simulink model "Regelkreis_T4_restored_from_autosave"  (R2025b)
settings: Solver=ode3  StartTime=0.0  StopTime=3  FixedStep=0.02  RelTol=1e-3
model workspace (MAT data in the model file):
  K_I = 1
  T_1 = [1 1]
settings Model: ExtModeTrigDuration=100  Creator=ofm31594  LastModifiedBy=janis

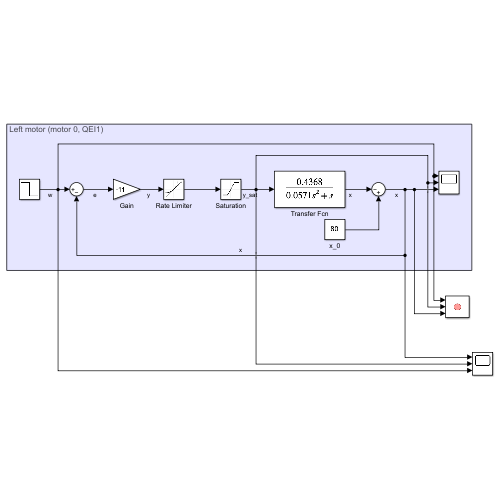
[thumbnail: Simulink's stored preview of the top-level diagram]
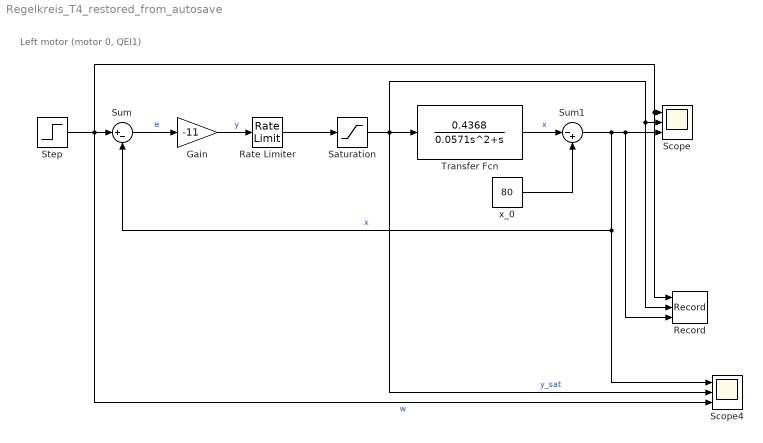
== system Regelkreis_T4_restored_from_autosave ==
  note: Left motor (motor 0, QEI1)
  Gain : Gain  Gain=-11
  Rate Limiter : RateLimiter  RisingSlewLimit=4/0.02  FallingSlewLimit=-20000  SampleTimeMode=inherited
  Record : Record  NumPorts=3.0  FileSettingsInternal="{\"entries\":[{\"content\":{\"excelSettings\":{\"content\":{},\"type\":\"Streamout.ExcelSettings\"},\"parquetSettings\":{\"content\":{},\"type\":\"Streamout.ParquetSettings\"}},\"type\":\"Streamout.FileSettingStorage\",\"uuid\":\"\"}],\"packageUris\":[\"http:\\/\\/schema.mathworks.com\\/mf0\\/streamout_blocks\\/R2020a\"],\"version\":\"1.0\"}"  FrameSettings=[0, 0, 0]  SignalsInternal="{\"entries\":[{\"content\":{\"signals\":[{\"content\":{\"blockPath\":[],\"dimensions\":[1,1],\"domain\":\"\",\"lineColor\":\"#edb120\",\"lineWidth\":2,\"plots\":[ 1 ],\"port\":1,\"sid\":[\"\"],\"signalID\":1,\"signalName\":\"w\"},\"type\":\"RecordBlkView.Signal\",\"uuid\":\"\"},{\"content\":{\"blockPath\":[],\"dimensions\":[1],\"domain\":\"\",\"lineColor\":\"#7e2f8e\",\"lineWidth\":2,\"plots\":[ 1 ],\"port\":2,\"sid\":[\"\"],\"signalID\":2,\"signalName\":\"y_sat\"},\"type\":\"RecordBlkView.Signal\",\"uuid\":\"\"},{\"content\":{\"blockPath\":[],\"dimensions\":[1],\"domain\":\"\",\"lineColor\":\"#77ac30\",\"lineWidth\":2,\"plots\":[ 1 ],\"port\":3,\"sid\":[\"\"],\"signalID\":3,\"signalName\":\"x\"},\"type\":\"RecordBlkView.Signal\",\"uuid\":\"\"}]},\"type\":\"RecordBlkView.InputSignals\",\"uuid\":\"\"}],\"packageUris\":[\"http:\\/\\/schema.mathworks.com\\/mf0\\/streamout_blocks\\/R2020a\"],\"version\":\"1.0\"}"  VisualizationBindings="{\"sparklinesplugin\":{\"info\":[{\"bindingParametersList\":[],\"subplotID\":1}]}}"
  Saturation : Saturate  UpperLimit=100  LowerLimit=-100
  Scope : Scope  NumInputPorts=3
      settings: ActiveDisplayYMinimum=-115.35662128410816  ActiveDisplayYMaximum=123.92851347601201
  Scope4 : Scope  NumInputPorts=3
      settings: ActiveDisplayYMinimum=-12.506652917821803  ActiveDisplayYMaximum=112.50073921309131  DataLoggingVariableName=ScopeData4
  Step : Step  Time=0.5000  Before=80  After=25  VectorParams1D=off  ZeroCross=off
  Sum : Sum  Inputs=|+-
  Sum1 : Sum  Inputs=|-+
  Transfer Fcn : TransferFcn  Numerator=0.4368  Denominator="[ 0.0571 1  0]"
  x_0 : Constant  Value=80
  wires:
  Sum/1 -> Gain/1  "e"
  Gain/1 -> Rate Limiter/1  "y"
  Step/1 -> Scope4/3, Record/1, Scope/1, Sum/1  "w"
  Sum1/1 -> Scope4/1, Sum/2, Record/3, Scope/3  "x"
  Transfer Fcn/1 -> Sum1/1  "x"
  x_0/1 -> Sum1/2
  Rate Limiter/1 -> Saturation/1
  Saturation/1 -> Scope4/2, Record/2, Scope/2, Transfer Fcn/1  "y_sat"
